simulink model "system_simulation_training_creator1"  (R2025b)
settings: Solver=FixedStepAuto  StartTime=0.0  StopTime=10  FixedStep=Ts  RelTol=1e-3
undefined symbols (not defined in the file or in its folder): commande_system, Ts
settings Model: Creator=Max  LastModifiedBy=strig
settings SolverCC: AlgebraicLoopSolver=TrustRegion
settings DebuggingCC: UnconnectedInputMsg=warning  UnconnectedOutputMsg=warning  UnconnectedLineMsg=warning
settings ModelReferenceCC: EnableRefExpFcnMdlSchedulingChecks=on
settings RTWCC: GPUComputeCapability=3.5

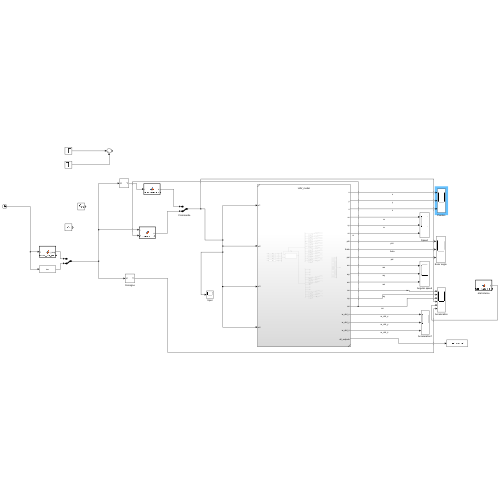
[thumbnail: Simulink's stored preview of the top-level diagram]
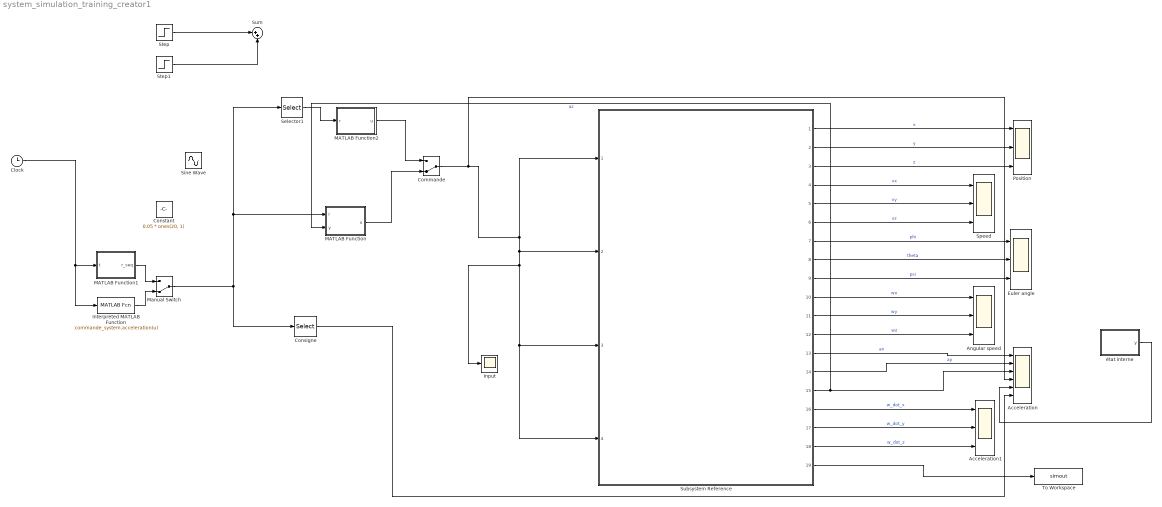
== system system_simulation_training_creator1 ==
  Acceleration : Scope  NumInputPorts=6
      settings: ActiveDisplayYMinimum=-13.59687263842237  ActiveDisplayYMaximum=10.248111830599871
  Acceleration1 : Scope  NumInputPorts=3
      settings: ActiveDisplayYMinimum=-40.918121722117149  ActiveDisplayYMaximum=44.001627281329164  DataLoggingVariableName=ScopeData2
  Angular speed : Scope  NumInputPorts=3
      settings: ActiveDisplayYMinimum=-1  ActiveDisplayYMaximum=1  DataLoggingVariableName=ScopeData3
  Clock : Clock
  Commande : ManualSwitch  CurrentSetting=0
  Consigne : Selector  InputPortWidth=20  IndexOptions=Index vector (dialog)  Indices=1  OutputSizes=1
  Constant : Constant  Value=0.05 * ones(20, 1)
  Euler angle : Scope  NumInputPorts=3
      settings: ActiveDisplayYMinimum=-1695.66598  ActiveDisplayYMaximum=1344.64163  DataLoggingVariableName=ScopeData4
  Input : Scope
      settings: ActiveDisplayYMinimum=0.31307209732175734  ActiveDisplayYMaximum=0.47677050883904804  DataLoggingVariableName=ScopeData5
  Interpreted MATLAB Function : MATLABFcn  MATLABFcn=commande_system.acceleration(u)
  MATLAB Function : MATLAB Function  TreatAsAtomicUnit=on
  MATLAB Function1 : MATLAB Function  TreatAsAtomicUnit=on
  MATLAB Function2 : MATLAB Function  TreatAsAtomicUnit=on
  Manual Switch : ManualSwitch  CurrentSetting=0
  Position : Scope  NumInputPorts=3
      settings: ActiveDisplayYMinimum=-7.0564531577369323  ActiveDisplayYMaximum=0.78348256156553819  DataLoggingVariableName=ScopeData6
  Selector1 : Selector  InputPortWidth=20  IndexOptions=Index vector (dialog)  Indices=1  OutputSizes=1
  Sine Wave : Sin  SampleTime=0
  Speed : Scope  NumInputPorts=3
      settings: ActiveDisplayYMinimum=-2.0291599170695513  ActiveDisplayYMaximum=0.93228871088825449
  Step : Step  SampleTime=0
  Step1 : Step  Time=3  After=-2  SampleTime=0
  Subsystem Reference : Subsystem  ReferencedSubsystem=UAV_model
  Sum : Sum  Inputs=|++
  To Workspace : ToWorkspace  VariableName=simout  SaveFormat=Structure With Time  SampleTime=Ts
  état interne : MATLAB Function  TreatAsAtomicUnit=on
  wires:
  Subsystem Reference/18 -> Acceleration1/3  "w_dot_z"
  Subsystem Reference/12 -> Angular speed/3  "wz"
  Subsystem Reference/17 -> Acceleration1/2  "w_dot_y"
  Subsystem Reference/9 -> Euler angle/3  "psi"
  Subsystem Reference/8 -> Euler angle/2  "theta"
  Subsystem Reference/14 -> Acceleration/2  "ay"
  Subsystem Reference/10 -> Angular speed/1  "wx"
  Subsystem Reference/2 -> Position/2  "y"
  Subsystem Reference/13 -> Acceleration/1  "ax"
  Subsystem Reference/15 -> MATLAB Function/2(y), Acceleration/3  "az"
  Subsystem Reference/16 -> Acceleration1/1  "w_dot_x"
  Subsystem Reference/7 -> Euler angle/1  "phi"
  Subsystem Reference/19 -> To Workspace/1
  Subsystem Reference/1 -> Position/1  "x"
  Subsystem Reference/6 -> Speed/3  "vz"
  Subsystem Reference/4 -> Speed/1  "vx"
  Subsystem Reference/3 -> Position/3  "z"
  Subsystem Reference/5 -> Speed/2  "vy"
  Subsystem Reference/11 -> Angular speed/2  "wy"
  Step/1 -> Sum/1
  Step1/1 -> Sum/2
  Clock/1 -> Interpreted MATLAB Function/1, MATLAB Function1/1(t)
  Consigne/1 -> Acceleration/6
  Selector1/1 -> MATLAB Function2/1(r)
  MATLAB Function2/1(u) -> Commande/1
  Commande/1 -> Acceleration/4, Subsystem Reference/4, Subsystem Reference/3, Input/1, Subsystem Reference/2, Subsystem Reference/1
  MATLAB Function/1(u) -> Commande/2
  état interne/1(y) -> Acceleration/5
  Interpreted MATLAB Function/1 -> Manual Switch/2
  Manual Switch/1 -> MATLAB Function/1(r), Selector1/1, Consigne/1
  MATLAB Function1/1(r_seq) -> Manual Switch/1

== matlab function system_simulation_training_creator1/MATLAB Function1 ==
  data: t input; r_seq output
function r_seq = generate_sin_preview(t)
    % --- CHOIX DU SIGNAL (Modifier ici) ---
    % 'sinus'   : Génère une sinusoïde
    % 'echelon' : Génère un échelon unité
    type_signal = 'sinus'; 
    
    % Paramètres du système et de la consigne (à adapter)
    Ts = 0.05;    % Temps d'échantillonnage discret de votre MPC
    % coder.extrinsic('evalin');
    N = 20; % evalin('base', 'horizon_N');;       % Horizon de prédiction (nombre d'échantillons)
    A = 3;        % Amplitude du signal
    f = 0.2;        % Fréquence en Hz (pour la sinusoïde)
    t_start = 1.0; % Instant de début de l'échelon (en secondes)
    
    % Création du vecteur des N prochains instants (t, t+Ts, ..., t+(N-1)*Ts)
    t_future = t + (0:N-1)' * Ts; 
    
    % Génération du signal selon la condition
    if strcmp(type_signal, 'sinus')
        r_seq = A * sin(2 * pi * f * t_future);
    elseif strcmp(type_signal, 'echelon')
        % Échelon différé : 1 pour t_future >= t_start, sinon 0
        r_seq = A * double(t_future >= t_start);
    else
        error('Type de signal non reconnu. Choisissez ''sinus'' ou ''echelon''.');
    end
end

== matlab function system_simulation_training_creator1/MATLAB Function2 ==
  data: r input; u output
function u = linear_controller_block(r)
%#codegen
persistent controller

% Déclarer les fonctions MATLAB non générables en C comme extrinsèques
coder.extrinsic('evalin', 'step');

% Définir le type et la taille de la sortie Simulink
u = 0.0;

% Récupérer l'instance mpc_system du Workspace MATLAB au 1er pas de temps
if isempty(controller)
    controller = evalin('base', 'linear_system');
end

% Appeler la méthode step() à chaque pas de temps de simulation
u = step(controller, r);
end

== matlab function system_simulation_training_creator1/état interne ==
  data: y output
function y = mpc_state_block()
%#codegen
coder.extrinsic('mpc_internal_state');
y = 0.0;                     % type et taille de la sortie
y = mpc_internal_state();
end

== matlab function system_simulation_training_creator1/MATLAB Function ==
  data: r input; u output; y input
function u = mpc_controller_block(r,y)
%#codegen
persistent controller

coder.extrinsic('evalin', 'step');

u = 0.0;

if isempty(controller)
    controller = evalin('base', 'mpc_system');
end

u = step(controller, r, y);
end
